simulink model "fuselage_lib_example"  (R2018b)
settings: Solver=FixedStepAuto  StartTime=0.0  StopTime=100  FixedStep=0.01  RelTol=1e-3
values from neighbouring files (symbols this model uses):
  fuselage = fuselageSetAeroelasticity(fuselage,structure,true)    [fuselageCreate.m]    (also in fuselageCreateWithCpacs.m; fuselageSetAeroState.m = fuselageSetLocalInflow( fuselage, xyz_cg ); fuselageSetGeometry.m = fuselageSetGeometryWidthVisc(fuselage,xi_interp,interp_metho; fuselageSetGeometryFromCpacs.m = fuselageSetGeometryWidthVisc(fuselage,fuselage.params.xi_seg)
libraries: atmosphere_lib x1, fuselage_lib x1
settings Model: Creator=Yannic  LastModifiedBy=yannic

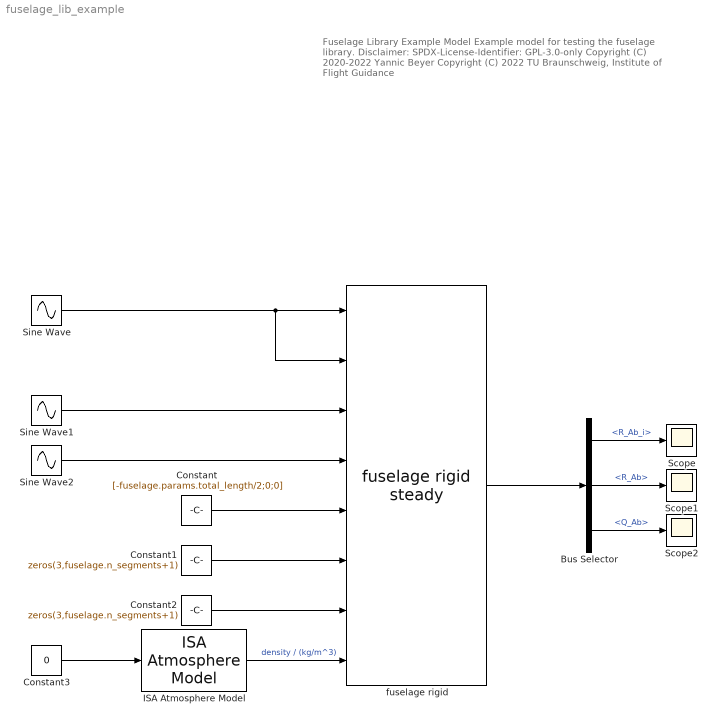
== system fuselage_lib_example ==
  note: Fuselage Library Example Model
      |
      | Example model for testing the fuselage library.
      |
      | Disclaimer:
      | SPDX-License-Identifier: GPL-3.0-only
      |
      | Copyright (C) 2020-2022 Yannic Beyer
      | Copyright (C) 2022 TU Braunschweig, Institute of Flight Guidance
  Bus Selector : BusSelector  OutputSignals=aero.R_Ab_i,aero.R_Ab,aero.Q_Ab
  Constant : Constant  Value=[-fuselage.params.total_length/2;0;0]  VectorParams1D=off
  Constant1 : Constant  Value=zeros(3,fuselage.n_segments+1)  VectorParams1D=off
  Constant2 : Constant  Value=zeros(3,fuselage.n_segments+1)  VectorParams1D=off
  Constant3 : Constant  Value=0  VectorParams1D=off
  ISA Atmosphere Model : atmosphere_lib/ISA Atmosphere Model
      settings: SourceProductName=LADAC
  Scope : Scope
  Scope1 : Scope
  Scope2 : Scope
  Sine Wave : Sin  Amplitude=0.1  Frequency=0.2  SampleTime=0
  Sine Wave1 : Sin  Amplitude=10  Bias=10  Frequency=0.1  SampleTime=0
  Sine Wave2 : Sin  Amplitude=ones(3,1)  Bias=zeros(3,1)  Frequency=[0.5;1;2]  SampleTime=0
  fuselage rigid : fuselage_lib/fuselage rigid steady  fuselage_struct=fuselage  fuselage_state_bus=fuselage_state_bus
      settings: SourceProductName=LADAC
  wires:
  Sine Wave/1 -> fuselage rigid/2, fuselage rigid/1
  Sine Wave1/1 -> fuselage rigid/3
  Sine Wave2/1 -> fuselage rigid/4
  fuselage rigid/1 -> Bus Selector/1
  Constant/1 -> fuselage rigid/5
  Constant1/1 -> fuselage rigid/6
  Constant2/1 -> fuselage rigid/7
  ISA Atmosphere Model/1 -> fuselage rigid/8  "density / (kg/m^3)"
  Constant3/1 -> ISA Atmosphere Model/1
  Bus Selector/1 -> Scope/1  "<R_Ab_i>"
  Bus Selector/2 -> Scope1/1  "<R_Ab>"
  Bus Selector/3 -> Scope2/1  "<Q_Ab>"
